simulink model "single_phase_afe_ideal"  (R2026a)
settings: Solver=ode23tb  StopTime=simlength  FixedStep=tc  MaxStep=glb_time.tc
values from neighbouring files (symbols this model uses):
  afe_ctrl = ctrl_afe_setup(glb_time.ts_afe, grid_emu.omega_grid_nom)    [init_model_legacy.m]
  frequency_set = 300    [init_model_legacy.m]
  glb_time = timing_setup(fpwm_afe, trgo_afe, fpwm_inv, trgo_inv, fpwm_single_phase_inv, trgo_single_phase_inv, fpwm_dab, trgo_dab,      fpwm_psfbc, trgo_psfbc, fpwm_isop_rail, trgo_isop_rail, fpwm_cllc, trgo_cllc, t_measure, tc_factor, tc_decimation, delay_pwm, dead_time_afe,      dead_time_inv, dead_time_single_phase_inv, dead_time_dab, dead_time_psfbc, dead_time_isop_rail, dead_time_cllc)    [init_model_legacy.m]
  grid_emu = grid_three_phase_emulator('Dyn11', delta_star, grid_nominal_power, application_voltage, us1, us2, fgrid,                  eq_grid_inductance, eq_grid_resistance, eta, ucc, i1m, p_iron, n1, n2, core_area, core_length, mur,                  up_xi_pu_ref, up_eta_pu_ref, un_xi_pu_ref, un_eta_pu_ref)    [init_model_legacy.m]
  heatsink = liquid_cooled_plate_2kw_setup(weight, no_weight, cp_al, heat_capacity_hs, thermal_conductivity_al,      Rth_switch_HA, Rth_mosfet_HA, Rth_diode_HA, Tambient, DThs_init)    [init_model_legacy.m]
  kepsilon = 2    [init_model_legacy.m]
  omega_set = frequency_set*2*pi    (= 1884.95559215)    [init_model_legacy.m]
  single_phase_inverter_ctrl = ctrl_single_phase_inverter_setup(glb_time.ts_inv, pres_ctrl.omega_set,      dqvector_pi.kp_inv, dqvector_pi.ki_inv, pres_ctrl.kp_rpi, pres_ctrl.ki_rpi, pres_ctrl.delta_rpi)    [init_model_legacy.m]
  Tambient = 40    [init_model_legacy.m]
  time_step_ref_1 = 0.025    [init_model_legacy.m]
  time_step_ref_2 = 0.5    [init_model_legacy.m]
  time_step_ref_3 = 1    [init_model_legacy.m]
  Vdc_nom = 400*1.35    (= 540)    [power_losses_calculation.m]
undefined symbols (not defined in the file or in its folder): delta_fht1, hwdata, igbt, Ld_fht1, magnitude, omega_fht1, ts_inv, Vac_FS, Xbez
libraries: fl_lib x116, nesl_utility x65, phase_shift_filter_ccaller x5, dq_vector_pi x4, igbt_simple_2th_lib x4, linear_double_integrator_observer_ccaller x3, lithium_ion_battery x1, dclink_for_two_levels x1, three_phase_voltage_with_frt_emulator x1, simulink x1, cstblocks_lti x1, single_phase_pwm_modulator x1
(part 2 of 6)

== system single_phase_afe_ideal/single_phase_inverter/single phase inverter control/pwm modulator ==
  vout : Inport
  Constant : Constant  Value=0
  Single phase two level PWM generator with global TRGO : single_phase_pwm_modulator/Single phase two level PWM generator with global TRGO  f=glb_time.fPWM_INV  m_up=0.98  m_low=0.02  dead_time=glb_time.dead_time_INV  pos_cmd_gate=18  neg_cmd_gate=-3  polarity=-1  tc=glb_time.tc  double_sampling=glb_time.TRGO_INV_double_update
  gate_cmds : Outport
  tag scope: TRGO_AFE_1=global
  wires:
  vout/1 -> Single phase two level PWM generator with global TRGO/3
  Constant/1 -> Single phase two level PWM generator with global TRGO/2
  Single phase two level PWM generator with global TRGO/2 -> gate_cmds/1
  Single phase two level PWM generator with global TRGO/1 -> [TRGO_AFE_1]
  [time_afe_module_1] -> Single phase two level PWM generator with global TRGO/1

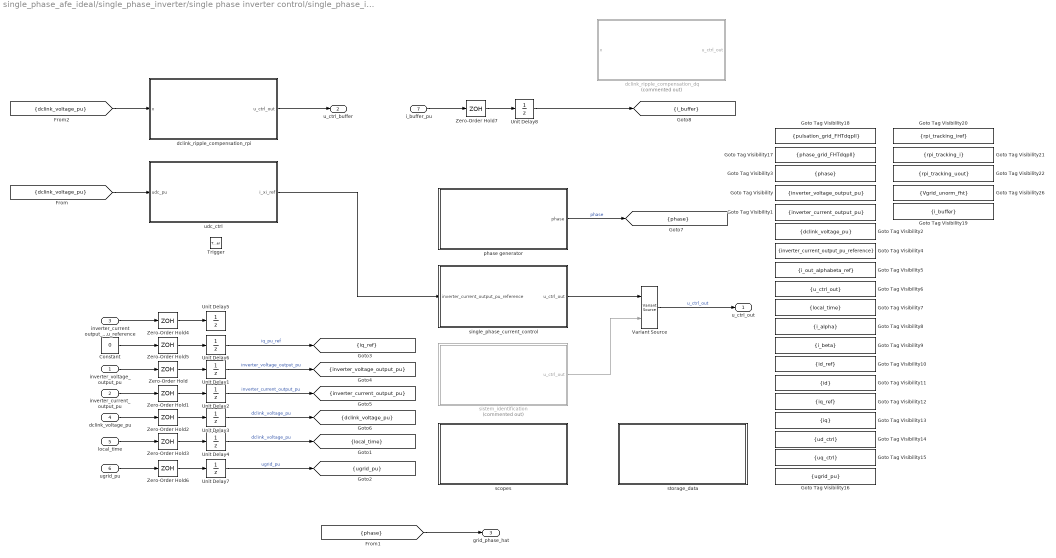
== system single_phase_afe_ideal/single_phase_inverter/single phase inverter control/single_phase_inverter_ctrl ==
  inverter_voltage_output_pu : Inport
  inverter_current_output_pu : Inport  Port=2
  inverter_current output_pu_reference : Inport  Port=3
  dclink_voltage_pu : Inport  Port=4
  local_time : Inport  Port=5
  ugrid_pu : Inport  Port=6
  i_buffer_pu : Inport  Port=7
  Trigger : TriggerPort  VariantControl=(inherit)  PortDimensions=1
  Constant : Constant  Value=0
  Goto Tag Visibility : GotoTagVisibility  GotoTag=inverter_voltage_output_pu
  Goto Tag Visibility1 : GotoTagVisibility  GotoTag=inverter_current_output_pu
  Goto Tag Visibility10 : GotoTagVisibility  GotoTag=id_ref
  Goto Tag Visibility11 : GotoTagVisibility  GotoTag=id
  Goto Tag Visibility12 : GotoTagVisibility  GotoTag=iq_ref
  Goto Tag Visibility13 : GotoTagVisibility  GotoTag=iq
  Goto Tag Visibility14 : GotoTagVisibility  GotoTag=ud_ctrl
  Goto Tag Visibility15 : GotoTagVisibility  GotoTag=uq_ctrl
  Goto Tag Visibility16 : GotoTagVisibility  GotoTag=ugrid_pu
  Goto Tag Visibility17 : GotoTagVisibility  GotoTag=phase_grid_FHTdqpll
  Goto Tag Visibility18 : GotoTagVisibility  GotoTag=pulsation_grid_FHTdqpll
  Goto Tag Visibility19 : GotoTagVisibility  GotoTag=i_buffer
  Goto Tag Visibility2 : GotoTagVisibility  GotoTag=dclink_voltage_pu
  Goto Tag Visibility20 : GotoTagVisibility  GotoTag=rpi_tracking_iref
  Goto Tag Visibility21 : GotoTagVisibility  GotoTag=rpi_tracking_i
  Goto Tag Visibility22 : GotoTagVisibility  GotoTag=rpi_tracking_uout
  Goto Tag Visibility26 : GotoTagVisibility  GotoTag=Vgrid_unorm_fht
  Goto Tag Visibility3 : GotoTagVisibility  GotoTag=phase
  Goto Tag Visibility4 : GotoTagVisibility  GotoTag=inverter_current_output_pu_reference
  Goto Tag Visibility5 : GotoTagVisibility  GotoTag=i_out_alphabeta_ref
  Goto Tag Visibility6 : GotoTagVisibility  GotoTag=u_ctrl_out
  Goto Tag Visibility7 : GotoTagVisibility  GotoTag=local_time
  Goto Tag Visibility8 : GotoTagVisibility  GotoTag=i_alpha
  Goto Tag Visibility9 : GotoTagVisibility  GotoTag=i_beta
  Unit Delay{1..8} (8 alike) : UnitDelay  SampleTime=-1
  Variant Source : VariantSource  VariantControls={system_identification_enable == 0, system_identification_enable == 1}
  Zero-Order Hold{,1..7} (8 alike) : ZeroOrderHold  SampleTime=-1
  dclink_ripple_compensation_dq : Subsystem  Commented=on
  dclink_ripple_compensation_rpi : Subsystem
  phase generator : Subsystem
  scopes : Subsystem
  single_phase_current_control : Subsystem
  sistem_identification : Subsystem  Commented=on
  storage_data : Subsystem
  udc_ctrl : Subsystem
  u_ctrl_out : Outport
  u_ctrl_buffer : Outport  Port=2
  grid_phase_hat : Outport  Port=3
  tag scope: dclink_voltage_pu=scoped, i_buffer=scoped, inverter_current_output_pu=scoped, inverter_voltage_output_pu=scoped, iq_ref=scoped, local_time=scoped, phase=scoped, ugrid_pu=scoped
  wires:
  inverter_voltage_output_pu/1 -> Zero-Order Hold/1
  inverter_current_output_pu/1 -> Zero-Order Hold1/1
  dclink_voltage_pu/1 -> Zero-Order Hold2/1
  Unit Delay1/1 -> [inverter_voltage_output_pu]  "inverter_voltage_output_pu"
  Unit Delay2/1 -> [inverter_current_output_pu]  "inverter_current_output_pu"
  Unit Delay3/1 -> [dclink_voltage_pu]  "dclink_voltage_pu"
  phase generator/1(phase) -> [phase]  "phase"
  inverter_current output_pu_reference/1 -> Zero-Order Hold4/1
  single_phase_current_control/1(u_ctrl_out) -> Variant Source/1
  Variant Source/1 -> u_ctrl_out/1  "u_ctrl_out"
  sistem_identification/1(u_ctrl_out) -> Variant Source/2
  Zero-Order Hold/1 -> Unit Delay1/1
  Zero-Order Hold1/1 -> Unit Delay2/1
  Zero-Order Hold2/1 -> Unit Delay3/1
  Zero-Order Hold3/1 -> Unit Delay4/1
  Unit Delay4/1 -> [local_time]  "dclink_voltage_pu"
  local_time/1 -> Zero-Order Hold3/1
  Zero-Order Hold4/1 -> Unit Delay5/1
  Constant/1 -> Zero-Order Hold5/1
  Zero-Order Hold5/1 -> Unit Delay6/1
  Unit Delay6/1 -> [iq_ref]  "iq_pu_ref"
  ugrid_pu/1 -> Zero-Order Hold6/1
  Zero-Order Hold6/1 -> Unit Delay7/1
  Unit Delay7/1 -> [ugrid_pu]  "ugrid_pu"
  [dclink_voltage_pu] -> udc_ctrl/1(udc_pu)
  udc_ctrl/1(i_xi_ref) -> single_phase_current_control/1(inverter_current_output_pu_reference)
  [phase] -> grid_phase_hat/1
  [dclink_voltage_pu] -> dclink_ripple_compensation_rpi/1(x)
  dclink_ripple_compensation_rpi/1(u_ctrl_out) -> u_ctrl_buffer/1
  Zero-Order Hold7/1 -> Unit Delay8/1
  i_buffer_pu/1 -> Zero-Order Hold7/1
  Unit Delay8/1 -> [i_buffer]

== system single_phase_afe_ideal/single_phase_inverter/single_phase_inverter/single phase inverter ==
  gate_cmds : Inport
  three_phase_inverter_with_igbt_simple_2th : Subsystem
  uac_out(+) : PMIOPort  Side=Left
  uac_out(-) : PMIOPort  Port=2  Side=Left
  udc(+) : PMIOPort  Port=3  Side=Right
  udc(-) : PMIOPort  Port=4  Side=Right
  wires:
  gate_cmds/1 -> three_phase_inverter_with_igbt_simple_2th/1(gate_cmds)
  connections:
  udc(-)/RConn1 -- three_phase_inverter_with_igbt_simple_2th/LConn2
  udc(+)/RConn1 -- three_phase_inverter_with_igbt_simple_2th/LConn1
  uac_out(+)/RConn1 -- three_phase_inverter_with_igbt_simple_2th/RConn1
  uac_out(-)/RConn1 -- three_phase_inverter_with_igbt_simple_2th/RConn2

== system single_phase_afe_ideal/single_phase_inverter/single phase inverter control/single_phase_inverter_ctrl/dclink_ripple_compensation_dq ==
  x : Inport
  Subsystem : Subsystem
  alphabeta2dq : Subsystem
  dq2alphabeta : Subsystem
  dq_vector_pi : Subsystem
  dq_vector_pi1 : Subsystem
  phase_shift_method_ccaller : Subsystem
  u_ctrl_out : Outport
  wires:
  Subsystem/1(x_hat_ac) -> phase_shift_method_ccaller/1(x_in)  "udc_hat_pu"
  x/1 -> Subsystem/1(x)  "udc_pu"
  phase_shift_method_ccaller/1(x_out) -> alphabeta2dq/1(alpha)
  phase_shift_method_ccaller/2(y_out) -> alphabeta2dq/2(beta)
  alphabeta2dq/1("d ") -> dq_vector_pi/1(d)
  alphabeta2dq/2("q ") -> dq_vector_pi/2(q)
  dq_vector_pi/1(id_ref) -> dq_vector_pi1/1(id_ref)
  dq_vector_pi/2(iq_ref) -> dq_vector_pi1/2(iq_ref)
  dq_vector_pi1/1(ud_ctrl) -> dq2alphabeta/1(d)
  dq_vector_pi1/2(uq_ctrl) -> dq2alphabeta/2(q)
  dq2alphabeta/1(beta) -> u_ctrl_out/1

== system single_phase_afe_ideal/single_phase_inverter/single phase inverter control/single_phase_inverter_ctrl/dclink_ripple_compensation_rpi ==
  x : Inport
  alphabeta2dq : Subsystem
  dclink compensation : Scope  NumInputPorts=4
      settings: ActiveDisplayString=3  ActiveDisplayYMinimum=-0.23625291597998122  ActiveDisplayYMaximum=0.43484103537778063  DataLoggingVariableName=ScopeData11
  dclink compensation performance : Scope  NumInputPorts=4
      settings: ActiveDisplayString=3  ActiveDisplayYMinimum=0.96431297385248793  ActiveDisplayYMaximum=1.025890884184312  DataLoggingVariableName=ScopeData10
  dq2alphabeta : Subsystem
  dq_vector_pi : Subsystem
  dx_dt : Subsystem
  phase_shift_method_ccaller : Subsystem
  u_ctrl_out : Outport
  wires:
  dq2alphabeta/1(beta) -> u_ctrl_out/1, dclink compensation performance/1  "iref"
  dq_vector_pi/2(uq_ctrl) -> dclink compensation/4, dq2alphabeta/2(q)
  dq_vector_pi/1(ud_ctrl) -> dclink compensation/3, dq2alphabeta/1(d)
  alphabeta2dq/2("q ") -> dclink compensation/2, dq_vector_pi/2(q)
  alphabeta2dq/1("d ") -> dclink compensation/1, dq_vector_pi/1(d)
  phase_shift_method_ccaller/2(y_out) -> alphabeta2dq/2(beta)
  phase_shift_method_ccaller/1(x_out) -> alphabeta2dq/1(alpha)
  x/1 -> dx_dt/1(x), dclink compensation performance/3  "udc_pu"
  dx_dt/1(x_hat_ac) -> phase_shift_method_ccaller/1(x_in), dclink compensation performance/2  "udc_hat_pu"

== system single_phase_afe_ideal/single_phase_inverter/single phase inverter control/single_phase_inverter_ctrl/phase generator ==
  FHT-PLL : Subsystem
  FHTdqpll : Scope  NumInputPorts=2
      settings: ActiveDisplayYMinimum=-1.624956414103508  ActiveDisplayYMaximum=4.624995157122612  DataLoggingVariableName=ScopeData3
  phase : Outport
  tag scope: phase_grid_FHTdqpll=scoped, pulsation_grid_FHTdqpll=scoped
  wires:
  FHT-PLL/1(phase_grid_fht_pll) -> [phase_grid_FHTdqpll]
  FHT-PLL/2(omega_grid_fht_pll) -> [pulsation_grid_FHTdqpll]
  [ugrid_pu] -> FHT-PLL/1(ug_abc_pu)
  [phase_grid_FHTdqpll] -> FHTdqpll/1  "phase_grid_FHTdqpll"
  [pulsation_grid_FHTdqpll] -> FHTdqpll/2  "pulsation_grid_FHTdqpll"
  [phase_grid_FHTdqpll] -> phase/1

== system single_phase_afe_ideal/single_phase_inverter/single phase inverter control/single_phase_inverter_ctrl/scopes ==
  Bus Creator1 : BusCreator  Inputs=3
  Bus Creator2 : BusCreator  Inputs=2
  Bus Creator3 : BusCreator  Inputs=2
  Bus Creator4 : BusCreator  Inputs=2
  single phase inverter tracking current scope 1 : Scope  NumInputPorts=2
      settings: ActiveDisplayYMinimum=-1.23468017578125  ActiveDisplayYMaximum=1.23419189453125  DataLoggingVariableName=ScopeData12
  single phase inverter tracking current scope 2 : Scope  NumInputPorts=2
      settings: ActiveDisplayYMinimum=-1.2603759765625  ActiveDisplayYMaximum=1.2652587890625  DataLoggingVariableName=ScopeData2
  wires:
  Bus Creator1/1 -> single phase inverter tracking current scope 1/2  "is_tracking"
  [i_out_alphabeta_ref] -> Bus Creator1/2  "i_out_inverter_pu_ref"
  [inverter_current_output_pu] -> Bus Creator1/3  "inverter_current_output_pu"
  [inverter_voltage_output_pu] -> Bus Creator2/1  "inverter_voltage_output_pu"
  Bus Creator2/1 -> single phase inverter tracking current scope 1/1  "load"
  [inverter_current_output_pu_reference] -> Bus Creator1/1  "inverter_current_output_pu_reference"
  [inverter_current_output_pu] -> Bus Creator2/2  "inverter_current_output_pu"
  [u_ctrl_out] -> Bus Creator3/1  "u_ctrl_out"
  [inverter_voltage_output_pu] -> Bus Creator3/2  "inverter_voltage_output_pu"
  Bus Creator3/1 -> single phase inverter tracking current scope 2/2  "u_load"
  [inverter_current_output_pu] -> Bus Creator4/2  "inverter_current_output_pu"
  [i_out_alphabeta_ref] -> Bus Creator4/1  "i_out_alphabeta_ref"
  Bus Creator4/1 -> single phase inverter tracking current scope 2/1  "i_load"

== system single_phase_afe_ideal/single_phase_inverter/single phase inverter control/single_phase_inverter_ctrl/single_phase_current_control ==
  inverter_current_output_pu_reference : Inport
  current_reference_generation : Subsystem
  dqpi_current_controller : Subsystem
  u_ctrl_out : Outport
  tag scope: i_out_alphabeta_ref=scoped, inverter_current_output_pu_reference=scoped, u_ctrl_out=scoped
  wires:
  current_reference_generation/1(is_ref) -> [i_out_alphabeta_ref]  "i_out_inverter_pu_ref"
  dqpi_current_controller/1(u_out) -> u_ctrl_out/1, [u_ctrl_out]  "u_ctrl_out"
  [phase] -> current_reference_generation/2(phase)
  inverter_current_output_pu_reference/1 -> current_reference_generation/1(mag_ref), [inverter_current_output_pu_reference]
  current_reference_generation/2(id_ref) -> dqpi_current_controller/1(id_ref)

== system single_phase_afe_ideal/single_phase_inverter/single phase inverter control/single_phase_inverter_ctrl/sistem_identification ==
  open loop u/f : Subsystem
  u_ctrl_out : Outport
  wires:
  open loop u/f/1(u_out) -> u_ctrl_out/1  "u_ctrl_out"

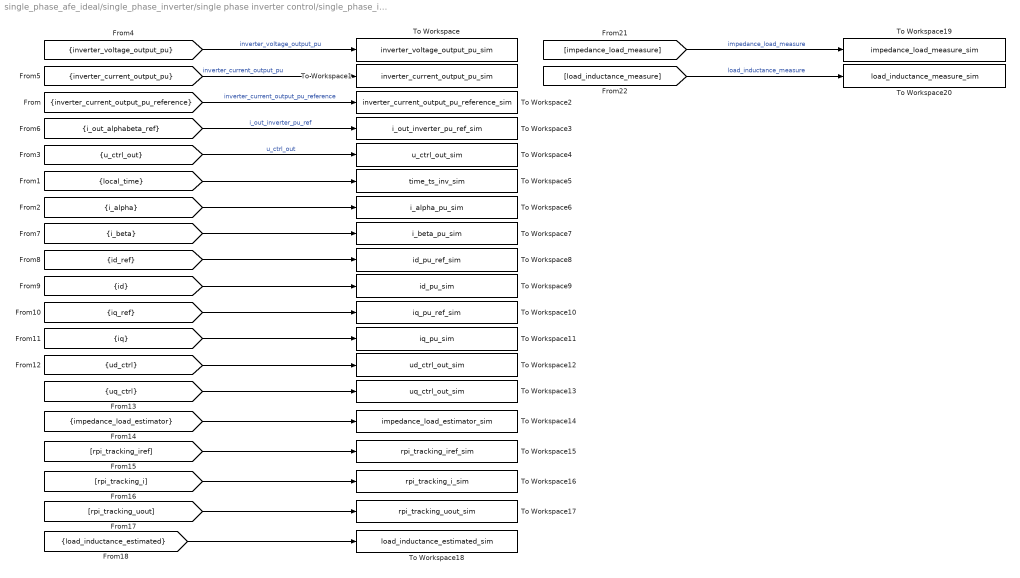
== system single_phase_afe_ideal/single_phase_inverter/single phase inverter control/single_phase_inverter_ctrl/storage_data ==
  To Workspace : ToWorkspace  VariableName=inverter_voltage_output_pu_sim  SampleTime=-1
      settings: MaxDataPoints=glb_time.Ns_inv  Save2DSignal=2-D array (concatenate along first dimension)
  To Workspace1 : ToWorkspace  VariableName=inverter_current_output_pu_sim  SampleTime=-1
      settings: MaxDataPoints=glb_time.Ns_inv  Save2DSignal=2-D array (concatenate along first dimension)
  To Workspace10 : ToWorkspace  VariableName=iq_pu_ref_sim  SampleTime=-1
      settings: MaxDataPoints=glb_time.Ns_inv  Save2DSignal=2-D array (concatenate along first dimension)
  To Workspace11 : ToWorkspace  VariableName=iq_pu_sim  SampleTime=-1
      settings: MaxDataPoints=glb_time.Ns_inv  Save2DSignal=2-D array (concatenate along first dimension)
  To Workspace12 : ToWorkspace  VariableName=ud_ctrl_out_sim  SampleTime=-1
      settings: MaxDataPoints=glb_time.Ns_inv  Save2DSignal=2-D array (concatenate along first dimension)
  To Workspace13 : ToWorkspace  VariableName=uq_ctrl_out_sim  SampleTime=-1
      settings: MaxDataPoints=glb_time.Ns_inv  Save2DSignal=2-D array (concatenate along first dimension)
  To Workspace14 : ToWorkspace  VariableName=impedance_load_estimator_sim  SampleTime=-1
      settings: MaxDataPoints=glb_time.Ns_inv  Save2DSignal=2-D array (concatenate along first dimension)
  To Workspace15 : ToWorkspace  VariableName=rpi_tracking_iref_sim  SampleTime=-1
      settings: MaxDataPoints=glb_time.Ns_inv  Save2DSignal=2-D array (concatenate along first dimension)
  To Workspace16 : ToWorkspace  VariableName=rpi_tracking_i_sim  SampleTime=-1
      settings: MaxDataPoints=glb_time.Ns_inv  Save2DSignal=2-D array (concatenate along first dimension)
  To Workspace17 : ToWorkspace  VariableName=rpi_tracking_uout_sim  SampleTime=-1
      settings: MaxDataPoints=glb_time.Ns_inv  Save2DSignal=2-D array (concatenate along first dimension)
  To Workspace18 : ToWorkspace  VariableName=load_inductance_estimated_sim  SampleTime=-1
      settings: MaxDataPoints=glb_time.Ns_inv  Save2DSignal=2-D array (concatenate along first dimension)
  To Workspace19 : ToWorkspace  VariableName=impedance_load_measure_sim  SampleTime=-1
      settings: MaxDataPoints=glb_time.Ns_inv  Save2DSignal=2-D array (concatenate along first dimension)
  To Workspace2 : ToWorkspace  VariableName=inverter_current_output_pu_reference_sim  SampleTime=-1
      settings: MaxDataPoints=glb_time.Ns_inv  Save2DSignal=2-D array (concatenate along first dimension)
  To Workspace20 : ToWorkspace  VariableName=load_inductance_measure_sim  SampleTime=-1
      settings: MaxDataPoints=glb_time.Ns_inv  Save2DSignal=2-D array (concatenate along first dimension)
  To Workspace3 : ToWorkspace  VariableName=i_out_inverter_pu_ref_sim  SampleTime=-1
      settings: MaxDataPoints=glb_time.Ns_inv  Save2DSignal=2-D array (concatenate along first dimension)
  To Workspace4 : ToWorkspace  VariableName=u_ctrl_out_sim  SampleTime=-1
      settings: MaxDataPoints=glb_time.Ns_inv  Save2DSignal=2-D array (concatenate along first dimension)
  To Workspace5 : ToWorkspace  VariableName=time_ts_inv_sim  SampleTime=-1
      settings: MaxDataPoints=glb_time.Ns_inv  Save2DSignal=2-D array (concatenate along first dimension)
  To Workspace6 : ToWorkspace  VariableName=i_alpha_pu_sim  SampleTime=-1
      settings: MaxDataPoints=glb_time.Ns_inv  Save2DSignal=2-D array (concatenate along first dimension)
  To Workspace7 : ToWorkspace  VariableName=i_beta_pu_sim  SampleTime=-1
      settings: MaxDataPoints=glb_time.Ns_inv  Save2DSignal=2-D array (concatenate along first dimension)
  To Workspace8 : ToWorkspace  VariableName=id_pu_ref_sim  SampleTime=-1
      settings: MaxDataPoints=glb_time.Ns_inv  Save2DSignal=2-D array (concatenate along first dimension)
  To Workspace9 : ToWorkspace  VariableName=id_pu_sim  SampleTime=-1
      settings: MaxDataPoints=glb_time.Ns_inv  Save2DSignal=2-D array (concatenate along first dimension)
  wires:
  [inverter_voltage_output_pu] -> To Workspace/1  "inverter_voltage_output_pu"
  [inverter_current_output_pu] -> To Workspace1/1  "inverter_current_output_pu"
  [inverter_current_output_pu_reference] -> To Workspace2/1  "inverter_current_output_pu_reference"
  [i_out_alphabeta_ref] -> To Workspace3/1  "i_out_inverter_pu_ref"
  [u_ctrl_out] -> To Workspace4/1  "u_ctrl_out"
  [local_time] -> To Workspace5/1
  [i_alpha] -> To Workspace6/1
  [i_beta] -> To Workspace7/1
  [id_ref] -> To Workspace8/1
  [id] -> To Workspace9/1
  [iq_ref] -> To Workspace10/1
  [iq] -> To Workspace11/1
  [ud_ctrl] -> To Workspace12/1
  [uq_ctrl] -> To Workspace13/1
  [impedance_load_estimator] -> To Workspace14/1
  [rpi_tracking_iref] -> To Workspace15/1
  [rpi_tracking_i] -> To Workspace16/1
  [rpi_tracking_uout] -> To Workspace17/1
  [load_inductance_estimated] -> To Workspace18/1
  [load_inductance_measure] -> To Workspace20/1  "load_inductance_measure"
  [impedance_load_measure] -> To Workspace19/1  "impedance_load_measure"

== system single_phase_afe_ideal/single_phase_inverter/single phase inverter control/single_phase_inverter_ctrl/udc_ctrl ==
  udc_pu : Inport
  1/Ti : Gain  Gain=afe_ctrl.kp_udc_ctrl  SaturateOnIntegerOverflow=on  OutDataTypeStr=Inherit: Same as input  ParamDataTypeStr=Inherit: Same as input
  Constant : Constant  Value=0
  Gain : Gain  Gain=-1
  Saturation : Saturate  UpperLimit=afe_ctrl.ixi_pos_ref_lim  LowerLimit=-afe_ctrl.ixi_pos_ref_lim
  Sum1 : Sum  Inputs=+++  SaturateOnIntegerOverflow=on
  Sum2 : Sum  Inputs=-+  SaturateOnIntegerOverflow=on
  Sum3 : Sum  Inputs=-+  SaturateOnIntegerOverflow=on
  Switch : Switch  Criteria=u2 > Threshold  SaturateOnIntegerOverflow=off  InputSameDT=off
  To Workspace1 : ToWorkspace  VariableName=udc_pu_sim_mod1  SampleTime=-1
      settings: MaxDataPoints=glb_time.Ns_afe
  To Workspace3 : ToWorkspace  VariableName=udc_pu_ref_sim_mod1  SampleTime=-1
      settings: MaxDataPoints=glb_time.Ns_afe
  Unit Delay4 : UnitDelay  SampleTime=-1
  discrete-time-low-pass-filter1 : discrete_time_low_pass_filter/discrete-time-low-pass-filter  tau=20e-3  ts=glb_time.ts_afe
  kp : Gain  Gain=afe_ctrl.ki_udc_ctrl*glb_time.ts_afe  SaturateOnIntegerOverflow=on  OutDataTypeStr=Inherit: Same as input  ParamDataTypeStr=Inherit: Same as input
  udc_norm_ref : Step  Time=1e-3  FinalValue=afe_ctrl.udc_norm_ref
  udc_tracking : Scope  NumInputPorts=3
      settings: ActiveDisplayYMinimum=-0.46728966593604021  ActiveDisplayYMaximum=2.2242301017706709  DataLoggingVariableName=ScopeData8
  i_xi_ref : Outport
  wires:
  1/Ti/1 -> Sum1/1, Sum3/1
  kp/1 -> Sum1/2
  Sum3/1 -> Unit Delay4/1
  Unit Delay4/1 -> Sum1/3
  udc_norm_ref/1 -> discrete-time-low-pass-filter1/1
  udc_pu/1 -> Sum2/1, To Workspace1/1, udc_tracking/2  "udc_pu"
  Sum2/1 -> kp/1, 1/Ti/1
  Sum1/1 -> Saturation/1
  [pwr_lim_enable] -> Switch/2
  Saturation/1 -> Switch/3
  Switch/1 -> Sum3/2, Gain/1
  Constant/1 -> Switch/1
  Gain/1 -> udc_tracking/3, i_xi_ref/1  "i_xi_ref"
  discrete-time-low-pass-filter1/1 -> To Workspace3/1, udc_tracking/1, Sum2/2  "udc_pu_ref"

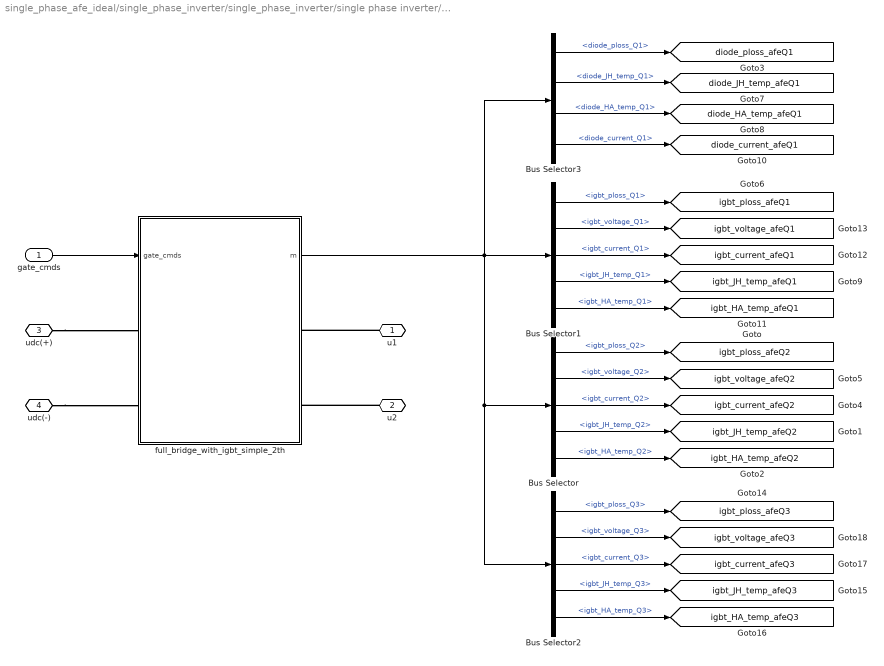
== system single_phase_afe_ideal/single_phase_inverter/single_phase_inverter/single phase inverter/three_phase_inverter_with_igbt_simple_2th ==
  gate_cmds : Inport
  Bus Selector : BusSelector  OutputSignals=module_1.igbt_ploss_Q2,module_1.igbt_voltage_Q2,module_1.igbt_current_Q2,module_1.igbt_JH_temp_Q2,module_1.igbt_HA_temp_Q2
  Bus Selector1 : BusSelector  OutputSignals=module_1.igbt_ploss_Q1,module_1.igbt_voltage_Q1,module_1.igbt_current_Q1,module_1.igbt_JH_temp_Q1,module_1.igbt_HA_temp_Q1
  Bus Selector2 : BusSelector  OutputSignals=module_2.igbt_ploss_Q3,module_2.igbt_voltage_Q3,module_2.igbt_current_Q3,module_2.igbt_JH_temp_Q3,module_2.igbt_HA_temp_Q3
  Bus Selector3 : BusSelector  OutputSignals=module_1.diode_ploss_Q1,module_1.diode_JH_temp_Q1,module_1.diode_HA_temp_Q1,module_1.diode_current_Q1
  full_bridge_with_igbt_simple_2th : Subsystem  mask{vce_sat_m=igbt.afe.Vce_sat, v_gamma_m=igbt.afe.Vdon_diode, Vth_gate_m=igbt.afe.Vth, Vth_gate_hyst_m=0.85, Eon_m=igbt.afe.Eon*1000, Eoff_m=igbt.afe.Eoff*1000, Err_m=igbt.afe.Erec*1000, Ic_ref_m=igbt.afe.Ion_sw_losses, Vdc_ref_m=igbt.afe.Voff_sw_losses, Vblock_Errf_m=50, rce_on_m=igbt.afe.Rce_on*1000, rd_on_m=igbt.afe.Rdon_diode*1000, Gce_off_m=1e-6, time_constant_edge_m=glb_time.tc, time_constant_ploss_m=1e3, Csnubber_m=igbt.afe.Csnubber_zvs, Rsnubber_m=igbt.afe.Rsnubber_zvs, rth_switch_JH_m=igbt.afe.Rth_switch_JH, rth_switch_HA_m=heatsink.Rth_switch_HA, rth_diode_JH_m=igbt.afe.Rth_diode_JH, rth_diode_HA_m=heatsink.Rth_diode_HA, JunctionTermalMass_m=igbt.afe.JunctionTermalMass, Tambient_m=Tambient, mass_heatsink_m=heatsink.no_weight, specific_heat_m=heatsink.cp}
      mask prompts: vce_sat_m "Collector-emitter on-stage voltage [V]"; v_gamma_m "Diode forward voltage [V]"; Vth_gate_m "Gate-emitter threshold voltage [V]"; Vth_gate_hyst_m "Half hysteresis band for the switching events [V]"; Eon_m "Turn-on energy at Ic_ref, Vdc_ref [mJ]"; Eoff_m "Turn-off energy at Ic_ref, Vdc_ref [mJ]"; Err_m "Reverse recovery energy at Ic_ref, Vdc_ref [mJ]"; Ic_ref_m "Reference current of the energies [A]"; Vdc_ref_m "Reference voltage of the energies [V]"; Vblock_Errf_m "V block Err"; rce_on_m "IGBT on-state series resistance [mOhm]"; rd_on_m "Diode series resistance [mOhm]"; Gce_off_m "Off-state conductance [1/Ohm]"; time_constant_edge_m "Sample&hold time constant (<< on-time) [us]"; time_constant_ploss_m "Loss averaging time constant (2-5 x Tsw) [us]"; Csnubber_m "Csnubber [F]"; Rsnubber_m "Rsnubber [Ohm]"; rth_switch_JH_m "Thermal impedance Junction-heatsink switch [K/W]"; rth_switch_HA_m "Thermal impedance heatsink-ambient switch[K/W]"; rth_diode_JH_m "Thermal impedance Junction-heatsink diode [K/W]"; rth_diode_HA_m "Thermal impedance heatsink-ambient diode [K/W]"; JunctionTermalMass_m "Junction Thermal Mass [J/K]"; Tambient_m "Ambient temperature [degC]"; mass_heatsink_m "Mass heatsink [kg]"; specific_heat_m "Specific heat capacity of the heatsink [J/K/Kg]"
  u1 : PMIOPort  Side=Right
  u2 : PMIOPort  Port=2  Side=Right
  udc(+) : PMIOPort  Port=3  Side=Left
  udc(-) : PMIOPort  Port=4  Side=Left
  tag scope: diode_HA_temp_afeQ1=global, diode_JH_temp_afeQ1=global, diode_current_afeQ1=global, diode_ploss_afeQ1=global, igbt_HA_temp_afeQ1=global, igbt_HA_temp_afeQ2=global, igbt_HA_temp_afeQ3=global, igbt_JH_temp_afeQ1=global, igbt_JH_temp_afeQ2=global, igbt_JH_temp_afeQ3=global, igbt_current_afeQ1=global, igbt_current_afeQ2=global, igbt_current_afeQ3=global, igbt_ploss_afeQ1=global, igbt_ploss_afeQ2=global, igbt_ploss_afeQ3=global, igbt_voltage_afeQ1=global, igbt_voltage_afeQ2=global, igbt_voltage_afeQ3=global
  wires:
  gate_cmds/1 -> full_bridge_with_igbt_simple_2th/1(gate_cmds)
  Bus Selector3/3 -> [diode_HA_temp_afeQ1]  "<diode_HA_temp_Q1>"
  Bus Selector/1 -> [igbt_ploss_afeQ2]  "<igbt_ploss_Q2>"
  Bus Selector3/2 -> [diode_JH_temp_afeQ1]  "<diode_JH_temp_Q1>"
  Bus Selector1/2 -> [igbt_voltage_afeQ1]  "<igbt_voltage_Q1>"
  Bus Selector/2 -> [igbt_voltage_afeQ2]  "<igbt_voltage_Q2>"
  Bus Selector/5 -> [igbt_HA_temp_afeQ2]  "<igbt_HA_temp_Q2>"
  Bus Selector2/5 -> [igbt_HA_temp_afeQ3]  "<igbt_HA_temp_Q3>"
  Bus Selector2/2 -> [igbt_voltage_afeQ3]  "<igbt_voltage_Q3>"
  Bus Selector/4 -> [igbt_JH_temp_afeQ2]  "<igbt_JH_temp_Q2>"
  Bus Selector1/4 -> [igbt_JH_temp_afeQ1]  "<igbt_JH_temp_Q1>"
  Bus Selector3/1 -> [diode_ploss_afeQ1]  "<diode_ploss_Q1>"
  Bus Selector2/4 -> [igbt_JH_temp_afeQ3]  "<igbt_JH_temp_Q3>"
  Bus Selector2/3 -> [igbt_current_afeQ3]  "<igbt_current_Q3>"
  full_bridge_with_igbt_simple_2th/1(m) -> Bus Selector2/1, Bus Selector/1, Bus Selector3/1, Bus Selector1/1
  Bus Selector1/3 -> [igbt_current_afeQ1]  "<igbt_current_Q1>"
  Bus Selector/3 -> [igbt_current_afeQ2]  "<igbt_current_Q2>"
  Bus Selector1/5 -> [igbt_HA_temp_afeQ1]  "<igbt_HA_temp_Q1>"
  Bus Selector2/1 -> [igbt_ploss_afeQ3]  "<igbt_ploss_Q3>"
  Bus Selector1/1 -> [igbt_ploss_afeQ1]  "<igbt_ploss_Q1>"
  Bus Selector3/4 -> [diode_current_afeQ1]  "<diode_current_Q1>"
  connections:
  u1/RConn1 -- full_bridge_with_igbt_simple_2th/RConn1
  u2/RConn1 -- full_bridge_with_igbt_simple_2th/RConn2
  udc(-)/RConn1 -- full_bridge_with_igbt_simple_2th/LConn2
  udc(+)/RConn1 -- full_bridge_with_igbt_simple_2th/LConn1

== system single_phase_afe_ideal/single_phase_inverter/single phase inverter control/single_phase_inverter_ctrl/dclink_ripple_compensation_dq/Subsystem ==
  x : Inport
  Gain1 : Gain  Gain=1/afe_ctrl.omega_base
  Terminator : Terminator
  linear_double_integrator_observer_ccaller : linear_double_integrator_observer_ccaller/linear_double_integrator_observer_ccaller  kx_m=afe_ctrl.di_obs.ktheta  kv_m=afe_ctrl.di_obs.komega  ts_m=glb_time.ts_afe  time_release=0.05  instance=1  tc_m=-1
  x_hat_ac : Outport
  wires:
  linear_double_integrator_observer_ccaller/2 -> Gain1/1
  linear_double_integrator_observer_ccaller/1 -> Terminator/1  "x_hat"
  x/1 -> linear_double_integrator_observer_ccaller/1
  Gain1/1 -> x_hat_ac/1  "x_hat_ac"

== system single_phase_afe_ideal/single_phase_inverter/single phase inverter control/single_phase_inverter_ctrl/dclink_ripple_compensation_dq/alphabeta2dq ==
  alpha : Inport
  beta : Inport  Port=2
  Gain : Gain  Gain=2
  MATLAB Function : MATLAB Function  TreatAsAtomicUnit=on
  "d " : Outport  VectorParamsAs1DForOutWhenUnconnected=off
  "q " : Outport  Port=2  VectorParamsAs1DForOutWhenUnconnected=off
  wires:
  alpha/1 -> MATLAB Function/1(alpha)
  beta/1 -> MATLAB Function/2(beta)
  MATLAB Function/1(d) -> "d "/1
  MATLAB Function/2(q) -> "q "/1
  [phase] -> Gain/1
  Gain/1 -> MATLAB Function/3(phase)

== system single_phase_afe_ideal/single_phase_inverter/single phase inverter control/single_phase_inverter_ctrl/dclink_ripple_compensation_dq/dq2alphabeta ==
  d : Inport
  q : Inport  Port=2
  Gain : Gain  Gain=2
  MATLAB Function : MATLAB Function  TreatAsAtomicUnit=on
  beta : Outport  VectorParamsAs1DForOutWhenUnconnected=off
  wires:
  d/1 -> MATLAB Function/1(d)
  q/1 -> MATLAB Function/2(q)
  [phase] -> Gain/1
  Gain/1 -> MATLAB Function/3(phase)
  MATLAB Function/2(beta) -> beta/1

== system single_phase_afe_ideal/single_phase_inverter/single phase inverter control/single_phase_inverter_ctrl/dclink_ripple_compensation_dq/dq_vector_pi ==
  d : Inport
  q : Inport  Port=2
  Constant : Constant
  Constant1 : Constant  Value=0
  Constant2 : Constant  Value=0
  Gain : Gain
  Gain1 : Gain
  dq_vector_pi : dq_vector_pi/dq_vector_pi  kp=0.5  ki=18  ts=glb_time.ts_afe  lim_ctrl_out=1  CTRPIFF_CLIP_RELEASE=CTRPIFF_CLIP_RELEASE
  id_ref : Outport
  iq_ref : Outport  Port=2
  wires:
  dq_vector_pi/1 -> Gain/1  "ud_ctrl"
  q/1 -> dq_vector_pi/4
  d/1 -> dq_vector_pi/2
  dq_vector_pi/2 -> Gain1/1  "uq_ctrl"
  Constant/1 -> dq_vector_pi/5
  Constant1/1 -> dq_vector_pi/3
  Constant2/1 -> dq_vector_pi/1
  Gain/1 -> id_ref/1
  Gain1/1 -> iq_ref/1

== system single_phase_afe_ideal/single_phase_inverter/single phase inverter control/single_phase_inverter_ctrl/dclink_ripple_compensation_dq/dq_vector_pi1 ==
  id_ref : Inport
  iq_ref : Inport  Port=2
  Constant : Constant
  Subsystem : Subsystem
  alphabeta2dq : Subsystem
  dclink compensation performance : Scope  NumInputPorts=4
      settings: ActiveDisplayYMinimum=-0.18239860340715844  ActiveDisplayYMaximum=0.1141178098290834  DataLoggingVariableName=ScopeData9
  dq_vector_pi : dq_vector_pi/dq_vector_pi  kp=single_phase_inverter_ctrl.kp_inv  ki=single_phase_inverter_ctrl.ki_inv  ts=glb_time.ts_inv  lim_ctrl_out=single_phase_inverter_ctrl.u_lim  CTRPIFF_CLIP_RELEASE=CTRPIFF_CLIP_RELEASE
  phase_shift_method_ccaller : Subsystem
  ud_ctrl : Outport
  uq_ctrl : Outport  Port=2
  wires:
  id_ref/1 -> dclink compensation performance/1, dq_vector_pi/1  "id_ref"
  iq_ref/1 -> dq_vector_pi/3, dclink compensation performance/3  "iq_ref"
  dq_vector_pi/1 -> ud_ctrl/1  "ud_ctrl"
  dq_vector_pi/2 -> uq_ctrl/1  "uq_ctrl"
  phase_shift_method_ccaller/1(x_out) -> alphabeta2dq/1(alpha)
  Subsystem/1(x_hat_ac) -> phase_shift_method_ccaller/1(x_in)  "udc_hat_pu"
  phase_shift_method_ccaller/2(y_out) -> alphabeta2dq/2(beta)
  alphabeta2dq/1("d ") -> dclink compensation performance/2, dq_vector_pi/2
  alphabeta2dq/2("q ") -> dclink compensation performance/4, dq_vector_pi/4
  Constant/1 -> dq_vector_pi/5
  [i_buffer] -> Subsystem/1(x)

== system single_phase_afe_ideal/single_phase_inverter/single phase inverter control/single_phase_inverter_ctrl/dclink_ripple_compensation_dq/phase_shift_method_ccaller ==
  x_in : Inport
  Gain : Gain  Gain=-1
  phase_shift_filter_ccaller : phase_shift_filter_ccaller/phase_shift_filter_ccaller  freq_m=2*frequency_set  ts_m=glb_time.ts_inv  scaling_m=1  reset_time_release=0.025  instance=1  tc_m=-1
  x_out : Outport
  y_out : Outport  Port=2
  wires:
  phase_shift_filter_ccaller/1 -> Gain/1
  Gain/1 -> y_out/1  "y"
  x_in/1 -> x_out/1, phase_shift_filter_ccaller/1

== system single_phase_afe_ideal/single_phase_inverter/single phase inverter control/single_phase_inverter_ctrl/dclink_ripple_compensation_rpi/alphabeta2dq ==
  alpha : Inport
  beta : Inport  Port=2
  Gain : Gain  Gain=2
  MATLAB Function : MATLAB Function  TreatAsAtomicUnit=on
  "d " : Outport  VectorParamsAs1DForOutWhenUnconnected=off
  "q " : Outport  Port=2  VectorParamsAs1DForOutWhenUnconnected=off
  wires:
  Gain/1 -> MATLAB Function/3(phase)
  [phase] -> Gain/1
  MATLAB Function/2(q) -> "q "/1
  MATLAB Function/1(d) -> "d "/1
  beta/1 -> MATLAB Function/2(beta)
  alpha/1 -> MATLAB Function/1(alpha)

== system single_phase_afe_ideal/single_phase_inverter/single phase inverter control/single_phase_inverter_ctrl/dclink_ripple_compensation_rpi/dq2alphabeta ==
  d : Inport
  q : Inport  Port=2
  Gain : Gain  Gain=2
  Gain1 : Gain
  Gain2 : Gain
  MATLAB Function : MATLAB Function  TreatAsAtomicUnit=on
  beta : Outport  VectorParamsAs1DForOutWhenUnconnected=off
  wires:
  Gain/1 -> MATLAB Function/3(phase)
  [phase] -> Gain/1
  q/1 -> MATLAB Function/2(q)
  d/1 -> MATLAB Function/1(d)
  MATLAB Function/1(alpha) -> Gain1/1
  MATLAB Function/2(beta) -> Gain2/1
  Gain2/1 -> beta/1

== system single_phase_afe_ideal/single_phase_inverter/single phase inverter control/single_phase_inverter_ctrl/dclink_ripple_compensation_rpi/dq_vector_pi ==
  d : Inport
  q : Inport  Port=2
  Constant : Constant
  Constant1 : Constant  Value=0
  Constant2 : Constant  Value=0
  Gain : Gain
  Gain1 : Gain
  dq_vector_pi : dq_vector_pi/dq_vector_pi  kp=2  ki=18  ts=glb_time.ts_afe  lim_ctrl_out=1  CTRPIFF_CLIP_RELEASE=CTRPIFF_CLIP_RELEASE
  ud_ctrl : Outport
  uq_ctrl : Outport  Port=2
  wires:
  Gain1/1 -> uq_ctrl/1
  Gain/1 -> ud_ctrl/1
  Constant2/1 -> dq_vector_pi/1
  Constant1/1 -> dq_vector_pi/3
  Constant/1 -> dq_vector_pi/5
  dq_vector_pi/2 -> Gain1/1  "uq_ctrl"
  d/1 -> dq_vector_pi/2
  q/1 -> dq_vector_pi/4
  dq_vector_pi/1 -> Gain/1  "ud_ctrl"

== system single_phase_afe_ideal/single_phase_inverter/single phase inverter control/single_phase_inverter_ctrl/dclink_ripple_compensation_rpi/dx_dt ==
  x : Inport
  Gain1 : Gain  Gain=1/afe_ctrl.omega_base
  Terminator : Terminator
  linear_double_integrator_observer_ccaller : linear_double_integrator_observer_ccaller/linear_double_integrator_observer_ccaller  kx_m=afe_ctrl.di_obs.ktheta  kv_m=afe_ctrl.di_obs.komega  ts_m=glb_time.ts_afe  time_release=0.05  instance=2  tc_m=-1
  x_hat_ac : Outport
  wires:
  Gain1/1 -> x_hat_ac/1  "x_hat_ac"
  x/1 -> linear_double_integrator_observer_ccaller/1
  linear_double_integrator_observer_ccaller/1 -> Terminator/1  "x_hat"
  linear_double_integrator_observer_ccaller/2 -> Gain1/1

== system single_phase_afe_ideal/single_phase_inverter/single phase inverter control/single_phase_inverter_ctrl/dclink_ripple_compensation_rpi/phase_shift_method_ccaller ==
  x_in : Inport
  Gain : Gain  Gain=-1
  phase_shift_filter_ccaller : phase_shift_filter_ccaller/phase_shift_filter_ccaller  freq_m=2*frequency_set  ts_m=glb_time.ts_afe  scaling_m=1  reset_time_release=0.025  instance=2  tc_m=-1
  x_out : Outport
  y_out : Outport  Port=2
  wires:
  x_in/1 -> phase_shift_filter_ccaller/1, x_out/1
  Gain/1 -> y_out/1  "y"
  phase_shift_filter_ccaller/1 -> Gain/1

== system single_phase_afe_ideal/single_phase_inverter/single phase inverter control/single_phase_inverter_ctrl/phase generator/FHT-PLL ==
  ug_abc_pu : Inport
  pll_stageA : Subsystem
  pll_stageB : Subsystem
  phase_grid_fht_pll : Outport
  omega_grid_fht_pll : Outport  Port=2
  wires:
  ug_abc_pu/1 -> pll_stageA/2(ug_abc_pu)
  pll_stageB/2(omega_grid_ddsrf_pll) -> omega_grid_fht_pll/1
  pll_stageA/1(u_grid_xi) -> pll_stageB/1(u_grid_pos_xi)  "u_grid_pos_xi"
  pll_stageA/2(u_grid_eta) -> pll_stageB/2(u_grid_pos_eta)  "u_grid_pos_eta"
  pll_stageB/1(gamma_grid_ddsrf_pll) -> phase_grid_fht_pll/1, pll_stageA/1(gamma_grid)

== system single_phase_afe_ideal/single_phase_inverter/single phase inverter control/single_phase_inverter_ctrl/single_phase_current_control/current_reference_generation ==
  mag_ref : Inport
  phase : Inport  Port=2
  Bus Creator : BusCreator  Inputs=2
  Product : Product
  Product1 : Product
  Sin : Trigonometry  Operator=cos
  Sin1 : Trigonometry
  is_ref : Outport
  id_ref : Outport  Port=2
  wires:
  Sin/1 -> Product/2
  phase/1 -> Sin1/1, Sin/1
  mag_ref/1 -> id_ref/1, Product1/1, Product/1
  Sin1/1 -> Product1/2
  Product/1 -> Bus Creator/1  "is_ref_alpha"
  Product1/1 -> Bus Creator/2  "is_ref_beta"
  Bus Creator/1 -> is_ref/1

== system single_phase_afe_ideal/single_phase_inverter/single phase inverter control/single_phase_inverter_ctrl/single_phase_current_control/dqpi_current_controller ==
  id_ref : Inport
  Bus Creator : BusCreator  Inputs=3
  Bus Creator1 : BusCreator  Inputs=3
  Constant : Constant
  Variant Source : VariantSource  VariantControls={use_current_controller_from_ccaller_mod1 == 0, use_current_controller_from_ccaller_mod1 == 1}
  Variant Source1 : VariantSource  VariantControls={use_current_controller_from_ccaller_mod1 == 0, use_current_controller_from_ccaller_mod1 == 1}
  alphabeta2dq : Subsystem
  dq2alphabeta : Subsystem
  dq_vector_pi : Subsystem
  dq_vector_pi_ccaller : Subsystem
  dq_vector_pi_tracking : Scope  NumInputPorts=2
      settings: ActiveDisplayYMinimum=-2.0908012345791049  ActiveDisplayYMaximum=2.0878875670210966  DataLoggingVariableName=ScopeData8
  i2alphabeta : Subsystem
  virtual_alpha_beta_currents : Scope  NumInputPorts=3
      settings: ActiveDisplayYMinimum=-1.2800386399030685  ActiveDisplayYMaximum=1.2757767885923386  DataLoggingVariableName=ScopeData2
  u_out : Outport
  tag scope: i_alpha=scoped, i_beta=scoped, id=scoped, id_ref=scoped, iq=scoped, ud_ctrl=scoped, uq_ctrl=scoped
  wires:
  dq2alphabeta/1(alpha) -> u_out/1
  id_ref/1 -> dq_vector_pi/1(id_ref), Bus Creator/1, [id_ref], dq_vector_pi_ccaller/2(id_ref)
  alphabeta2dq/1("d ") -> Bus Creator/2, [id], dq_vector_pi_ccaller/1(id), dq_vector_pi/2(id)  "id"
  alphabeta2dq/2("q ") -> dq_vector_pi/3(iq), Bus Creator1/2, [iq], dq_vector_pi_ccaller/3(iq)  "iq"
  [iq_ref] -> dq_vector_pi/4(iq_ref), dq_vector_pi_ccaller/4(iq_ref)
  Variant Source1/1 -> dq2alphabeta/2(q)  "ctrl_q_u"
  Variant Source/1 -> dq2alphabeta/1(d)  "ctrl_d_u"
  dq_vector_pi/1(ud_ctrl) -> Variant Source/1
  dq_vector_pi/2(uq_ctrl) -> Variant Source1/1
  Constant/1 -> dq_vector_pi_ccaller/5(udc_pu)
  dq_vector_pi_ccaller/1(ud_ctrl_out) -> [ud_ctrl], Variant Source/2
  dq_vector_pi_ccaller/2(uq_ctrl_out) -> [uq_ctrl], Variant Source1/2
  Bus Creator1/1 -> dq_vector_pi_tracking/2
  Bus Creator/1 -> dq_vector_pi_tracking/1
  [ud_ctrl] -> Bus Creator/3
  [uq_ctrl] -> Bus Creator1/3
  [iq_ref] -> Bus Creator1/1
  [inverter_current_output_pu] -> i2alphabeta/1(i_alpha), virtual_alpha_beta_currents/1  "i_load"
  i2alphabeta/1(i_alpha_out) -> alphabeta2dq/1(alpha), virtual_alpha_beta_currents/2, [i_alpha]  "i_alpha"
  i2alphabeta/2(i_beta_out) -> alphabeta2dq/2(beta), virtual_alpha_beta_currents/3, [i_beta]  "i_beta"

== system single_phase_afe_ideal/single_phase_inverter/single phase inverter control/single_phase_inverter_ctrl/sistem_identification/open loop u//f ==
  Constant2 : Constant  Value=0.75
  Data Store Memory : DataStoreMemory  DataStoreName=u_test  WriteAfterWriteMsg=warning  ShowAdditionalParam=off
  Data Store Read1 : DataStoreRead  DataStoreName=u_test  DataStoreElements=u_test  IndexOptions=Index vector (dialog)  Indices=1  OutputSizes=1
  Data Store Write : DataStoreWrite  DataStoreName=u_test  IndexOptions=Index vector (dialog)  Indices=1  OutputSizes=1
  Gain1 : Gain  Gain=1/omega_set
  Gain2 : Gain  Gain=Vdc_nom/Vac_FS
  Gain3 : Gain  Gain=Xbez
  Product : Product  Inputs=*/
  Saturation : Saturate  UpperLimit=inf  LowerLimit=0.1
  dq2alphabeta : Subsystem
  first_harmonic_tracker : Subsystem  Commented=on
  i_alpha_beta_system_identification : Scope  NumInputPorts=4
      settings: ActiveDisplayYMinimum=1.5097956747477865  ActiveDisplayYMaximum=1.9442466663089897  DataLoggingVariableName=ScopeData2
  module : Subsystem
  phase_shift_filter_ccaller : phase_shift_filter_ccaller/phase_shift_filter_ccaller  Commented=on  freq_m=frequency_set  ts_m=ts_inv  scaling_m=phase_shift_filter_gain  reset_time_release=0.025  instance=1  tc_m=-1
  sogi_ccaller : Subsystem
  u_out : Outport
  tag scope: impedance_load_estimator=scoped, load_inductance_estimated=scoped
  wires:
  [inverter_current_output_pu] -> sogi_ccaller/1(input)  "i_alpha"
  dq2alphabeta/1(alpha) -> u_out/1
  Data Store Read1/1 -> Product/1
  Constant2/1 -> Data Store Write/1
  Saturation/1 -> Product/2
  module/1(i) -> Saturation/1  "Iload"
  Product/1 -> Gain2/1
  Gain1/1 -> [load_inductance_estimated], i_alpha_beta_system_identification/2  "Lload"
  sogi_ccaller/1(alpha) -> i_alpha_beta_system_identification/3, module/1(i_alpha)  "i_alpha_sogi"
  sogi_ccaller/2(beta) -> i_alpha_beta_system_identification/4, module/2(i_beta)  "i_beta_sogi"
  Gain2/1 -> Gain3/1
  Gain3/1 -> [impedance_load_estimator], i_alpha_beta_system_identification/1, Gain1/1  "Xload"

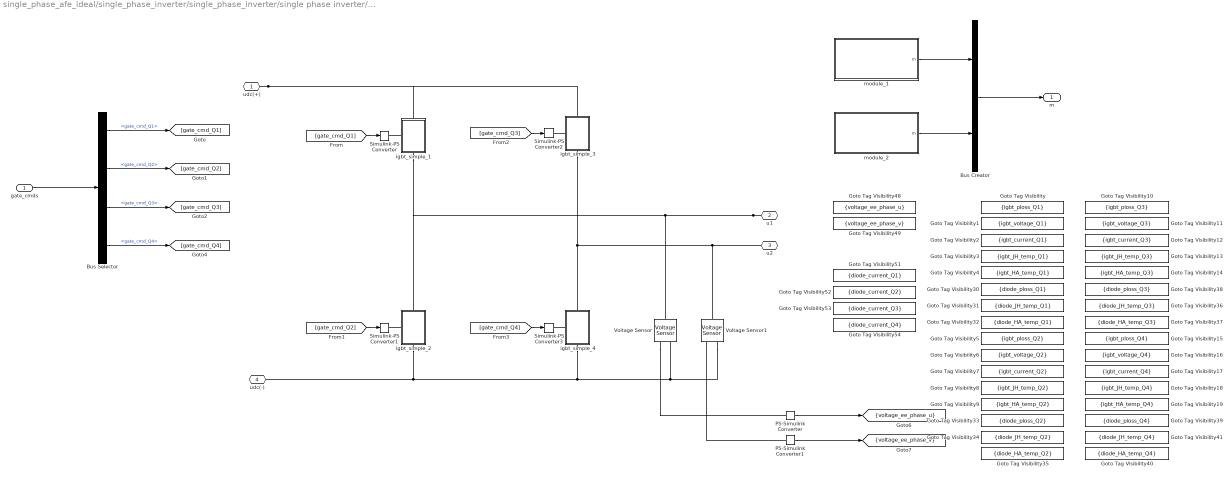
== system single_phase_afe_ideal/single_phase_inverter/single_phase_inverter/single phase inverter/three_phase_inverter_with_igbt_simple_2th/full_bridge_with_igbt_simple_2th ==
  gate_cmds : Inport
  Bus Creator : BusCreator  Inputs=2
  Bus Selector : BusSelector  OutputSignals=gate_cmd_Q1,gate_cmd_Q2,gate_cmd_Q3,gate_cmd_Q4
  Goto Tag Visibility : GotoTagVisibility  GotoTag=igbt_ploss_Q1
  Goto Tag Visibility1 : GotoTagVisibility  GotoTag=igbt_voltage_Q1
  Goto Tag Visibility10 : GotoTagVisibility  GotoTag=igbt_ploss_Q3
  Goto Tag Visibility11 : GotoTagVisibility  GotoTag=igbt_voltage_Q3
  Goto Tag Visibility12 : GotoTagVisibility  GotoTag=igbt_current_Q3
  Goto Tag Visibility13 : GotoTagVisibility  GotoTag=igbt_JH_temp_Q3
  Goto Tag Visibility14 : GotoTagVisibility  GotoTag=igbt_HA_temp_Q3
  Goto Tag Visibility15 : GotoTagVisibility  GotoTag=igbt_ploss_Q4
  Goto Tag Visibility16 : GotoTagVisibility  GotoTag=igbt_voltage_Q4
  Goto Tag Visibility17 : GotoTagVisibility  GotoTag=igbt_current_Q4
  Goto Tag Visibility18 : GotoTagVisibility  GotoTag=igbt_JH_temp_Q4
  Goto Tag Visibility19 : GotoTagVisibility  GotoTag=igbt_HA_temp_Q4
  Goto Tag Visibility2 : GotoTagVisibility  GotoTag=igbt_current_Q1
  Goto Tag Visibility3 : GotoTagVisibility  GotoTag=igbt_JH_temp_Q1
  Goto Tag Visibility30 : GotoTagVisibility  GotoTag=diode_ploss_Q1
  Goto Tag Visibility31 : GotoTagVisibility  GotoTag=diode_JH_temp_Q1
  Goto Tag Visibility32 : GotoTagVisibility  GotoTag=diode_HA_temp_Q1
  Goto Tag Visibility33 : GotoTagVisibility  GotoTag=diode_ploss_Q2
  Goto Tag Visibility34 : GotoTagVisibility  GotoTag=diode_JH_temp_Q2
  Goto Tag Visibility35 : GotoTagVisibility  GotoTag=diode_HA_temp_Q2
  Goto Tag Visibility36 : GotoTagVisibility  GotoTag=diode_JH_temp_Q3
  Goto Tag Visibility37 : GotoTagVisibility  GotoTag=diode_HA_temp_Q3
  Goto Tag Visibility38 : GotoTagVisibility  GotoTag=diode_ploss_Q3
  Goto Tag Visibility39 : GotoTagVisibility  GotoTag=diode_ploss_Q4
  Goto Tag Visibility4 : GotoTagVisibility  GotoTag=igbt_HA_temp_Q1
  Goto Tag Visibility40 : GotoTagVisibility  GotoTag=diode_HA_temp_Q4
  Goto Tag Visibility41 : GotoTagVisibility  GotoTag=diode_JH_temp_Q4
  Goto Tag Visibility48 : GotoTagVisibility  GotoTag=voltage_ee_phase_u
  Goto Tag Visibility49 : GotoTagVisibility  GotoTag=voltage_ee_phase_v
  Goto Tag Visibility5 : GotoTagVisibility  GotoTag=igbt_ploss_Q2
  Goto Tag Visibility51 : GotoTagVisibility  GotoTag=diode_current_Q1
  Goto Tag Visibility52 : GotoTagVisibility  GotoTag=diode_current_Q2
  Goto Tag Visibility53 : GotoTagVisibility  GotoTag=diode_current_Q3
  Goto Tag Visibility54 : GotoTagVisibility  GotoTag=diode_current_Q4
  Goto Tag Visibility6 : GotoTagVisibility  GotoTag=igbt_voltage_Q2
  Goto Tag Visibility7 : GotoTagVisibility  GotoTag=igbt_current_Q2
  Goto Tag Visibility8 : GotoTagVisibility  GotoTag=igbt_JH_temp_Q2
  Goto Tag Visibility9 : GotoTagVisibility  GotoTag=igbt_HA_temp_Q2
  PS-Simulink Converter : nesl_utility/PS-Simulink Converter  PhysicalDomain=network_engine_domain  SubClassName=ps_output  LeftPortType=input  RightPortType=output  PseudoPeriodic=off  Frequencies=[]  VectorFormat=1-D array  Unit=V  AffineConversion=off
  PS-Simulink Converter1 : nesl_utility/PS-Simulink Converter  PhysicalDomain=network_engine_domain  SubClassName=ps_output  LeftPortType=input  RightPortType=output  PseudoPeriodic=off  Frequencies=[]  VectorFormat=1-D array  Unit=V  AffineConversion=off
  Simulink-PS Converter{,1..3} (4 alike) : nesl_utility/Simulink-PS Converter  PhysicalDomain=network_engine_domain  SubClassName=ps_input  LeftPortType=input  RightPortType=output  PseudoPeriodic=off  Frequencies=[]  NoiseDistribution=none  NoiseParameters=[]  Unit=V  AffineConversion=off  FilteringAndDerivatives=provide  SimscapeFilterOrder=1  InputFilterTimeConstant=0.001  UdotUserProvided=0
  Voltage Sensor : fl_lib/Electrical/Electrical Sensors/Voltage Sensor
  Voltage Sensor1 : fl_lib/Electrical/Electrical Sensors/Voltage Sensor
  igbt_simple_1 : Subsystem
      settings: PortSchema="{\"entries\":[{\"content\":{\"sides\":[{\"content\":{\"connectorIds\":[\"LConn1\"]},\"type\":\"ConnectorPlacement.EquallySpacedRectSide\",\"uuid\":\"9277da8d-d460-43e6-8478-dd662f15d226\"},{\"content\":{\"connectorIds\":[],\"side\":\"RIGHT\"},\"type\":\"ConnectorPlacement.EquallySpacedRectSide\",\"uuid\":\"a7ece396-f1d9-4f4f-a05b-db1fc65d6e1d\"},{\"content\":{\"connectorIds\":[\"LConn2\"],\"side\":\"TOP\"},\"type\":\"ConnectorPlacement.EquallySpacedRectSide\",\"uuid\":\"fdd70777-e9cf-4317-afb6-cae87f75d5b0\"},{\"content\":{\"connectorIds\":[\"RConn1\"],\"side\":\"BOTTOM\"},\"type\":\"ConnectorPlacement.EquallySpacedRectSide\",\"uuid\":\"2353ed68-b1a1-4775-9ca9-31e268d5443b\"}]},\"type\":\"ConnectorPlacement.EquallySpacedConnector\",\"uuid\":\"d5479f4c-4e65-4791-adcb-73df11f88590\"}],\"packageUris\":[\"http://schema.mathworks.com/mf0/Connector/R2020b\"],\"version\":\"1.0\"}"
  igbt_simple_2 : Subsystem
      settings: PortSchema="{\"entries\":[{\"content\":{\"sides\":[{\"content\":{\"connectorIds\":[\"LConn1\"]},\"type\":\"ConnectorPlacement.EquallySpacedRectSide\",\"uuid\":\"9277da8d-d460-43e6-8478-dd662f15d226\"},{\"content\":{\"connectorIds\":[],\"side\":\"RIGHT\"},\"type\":\"ConnectorPlacement.EquallySpacedRectSide\",\"uuid\":\"a7ece396-f1d9-4f4f-a05b-db1fc65d6e1d\"},{\"content\":{\"connectorIds\":[\"LConn2\"],\"side\":\"TOP\"},\"type\":\"ConnectorPlacement.EquallySpacedRectSide\",\"uuid\":\"fdd70777-e9cf-4317-afb6-cae87f75d5b0\"},{\"content\":{\"connectorIds\":[\"RConn1\"],\"side\":\"BOTTOM\"},\"type\":\"ConnectorPlacement.EquallySpacedRectSide\",\"uuid\":\"2353ed68-b1a1-4775-9ca9-31e268d5443b\"}]},\"type\":\"ConnectorPlacement.EquallySpacedConnector\",\"uuid\":\"d5479f4c-4e65-4791-adcb-73df11f88590\"}],\"packageUris\":[\"http://schema.mathworks.com/mf0/Connector/R2020b\"],\"version\":\"1.0\"}"
  igbt_simple_3 : Subsystem
      settings: PortSchema="{\"entries\":[{\"content\":{\"sides\":[{\"content\":{\"connectorIds\":[\"LConn1\"]},\"type\":\"ConnectorPlacement.EquallySpacedRectSide\",\"uuid\":\"9277da8d-d460-43e6-8478-dd662f15d226\"},{\"content\":{\"connectorIds\":[],\"side\":\"RIGHT\"},\"type\":\"ConnectorPlacement.EquallySpacedRectSide\",\"uuid\":\"a7ece396-f1d9-4f4f-a05b-db1fc65d6e1d\"},{\"content\":{\"connectorIds\":[\"LConn2\"],\"side\":\"TOP\"},\"type\":\"ConnectorPlacement.EquallySpacedRectSide\",\"uuid\":\"fdd70777-e9cf-4317-afb6-cae87f75d5b0\"},{\"content\":{\"connectorIds\":[\"RConn1\"],\"side\":\"BOTTOM\"},\"type\":\"ConnectorPlacement.EquallySpacedRectSide\",\"uuid\":\"2353ed68-b1a1-4775-9ca9-31e268d5443b\"}]},\"type\":\"ConnectorPlacement.EquallySpacedConnector\",\"uuid\":\"d5479f4c-4e65-4791-adcb-73df11f88590\"}],\"packageUris\":[\"http://schema.mathworks.com/mf0/Connector/R2020b\"],\"version\":\"1.0\"}"
  igbt_simple_4 : Subsystem
      settings: PortSchema="{\"entries\":[{\"content\":{\"sides\":[{\"content\":{\"connectorIds\":[\"LConn1\"]},\"type\":\"ConnectorPlacement.EquallySpacedRectSide\",\"uuid\":\"9277da8d-d460-43e6-8478-dd662f15d226\"},{\"content\":{\"connectorIds\":[],\"side\":\"RIGHT\"},\"type\":\"ConnectorPlacement.EquallySpacedRectSide\",\"uuid\":\"a7ece396-f1d9-4f4f-a05b-db1fc65d6e1d\"},{\"content\":{\"connectorIds\":[\"LConn2\"],\"side\":\"TOP\"},\"type\":\"ConnectorPlacement.EquallySpacedRectSide\",\"uuid\":\"fdd70777-e9cf-4317-afb6-cae87f75d5b0\"},{\"content\":{\"connectorIds\":[\"RConn1\"],\"side\":\"BOTTOM\"},\"type\":\"ConnectorPlacement.EquallySpacedRectSide\",\"uuid\":\"2353ed68-b1a1-4775-9ca9-31e268d5443b\"}]},\"type\":\"ConnectorPlacement.EquallySpacedConnector\",\"uuid\":\"d5479f4c-4e65-4791-adcb-73df11f88590\"}],\"packageUris\":[\"http://schema.mathworks.com/mf0/Connector/R2020b\"],\"version\":\"1.0\"}"
  module_1 : Subsystem
  module_2 : Subsystem
  udc(+) : PMIOPort  Side=Left
  u1 : PMIOPort  Port=2  Side=Right
  u2 : PMIOPort  Port=3  Side=Right
  udc(-) : PMIOPort  Port=4  Side=Left
  m : Outport
  tag scope: voltage_ee_phase_u=scoped, voltage_ee_phase_v=scoped
  wires:
  module_1/1(m) -> Bus Creator/1
  Bus Creator/1 -> m/1
  module_2/1(m) -> Bus Creator/2
  PS-Simulink Converter1/1 -> [voltage_ee_phase_v]
  PS-Simulink Converter/1 -> [voltage_ee_phase_u]
  [gate_cmd_Q3] -> Simulink-PS Converter2/1
  [gate_cmd_Q4] -> Simulink-PS Converter3/1
  [gate_cmd_Q2] -> Simulink-PS Converter1/1
  [gate_cmd_Q1] -> Simulink-PS Converter/1
  gate_cmds/1 -> Bus Selector/1
  Bus Selector/4 -> [gate_cmd_Q4]  "<gate_cmd_Q4>"
  Bus Selector/3 -> [gate_cmd_Q3]  "<gate_cmd_Q3>"
  Bus Selector/2 -> [gate_cmd_Q2]  "<gate_cmd_Q2>"
  Bus Selector/1 -> [gate_cmd_Q1]  "<gate_cmd_Q1>"
  connections:
  PS-Simulink Converter1/LConn1 -- Voltage Sensor1/RConn1
  Voltage Sensor/RConn1 -- PS-Simulink Converter/LConn1
  u2/RConn1 -- igbt_simple_3/RConn1 -- igbt_simple_4/LConn2 -- Voltage Sensor1/LConn1
  Voltage Sensor1/RConn2 -- igbt_simple_4/RConn1 -- igbt_simple_2/RConn1 -- udc(-)/RConn1 -- Voltage Sensor/RConn2
  igbt_simple_4/LConn1 -- Simulink-PS Converter3/RConn1
  igbt_simple_3/LConn1 -- Simulink-PS Converter2/RConn1
  igbt_simple_2/LConn1 -- Simulink-PS Converter1/RConn1
  igbt_simple_1/LConn1 -- Simulink-PS Converter/RConn1
  udc(+)/RConn1 -- igbt_simple_3/LConn2 -- igbt_simple_1/LConn2
  u1/RConn1 -- igbt_simple_1/RConn1 -- igbt_simple_2/LConn2 -- Voltage Sensor/LConn1
